simulink model "tsc_lazo_cerrado"  (R2024a)
settings: Solver=ode15s  StartTime=0.0  StopTime=tm_final  MaxStep=tm_h  RelTol=1e-9  AbsTol=1e-11
model workspace (MAT data in the model file):
  tm_C1 = 1.87501784269e-05
  tm_C2 = 3.75003568539e-05
  tm_Cp = 2.89288467158e-06
  tm_L1 = 0.26018031666
  tm_L2 = 0.13009015833
  tm_R1 = 1.15690788571
  tm_R2 = 0.578453942857
  tm_Rb1 = 84640
  tm_Rb2 = 42320
  tm_Rp = 2.20064
  tm_a1 = 1
  tm_a2 = 0.03
  tm_a3 = 0.03
  tm_carga = [0 1e-05 2e-05 3e-05 4e-05 5e-05 6e-05 7e-05 8e-05 9e-05 0.0001 0.00011 ... (160002 elements, 80001x2)]
  tm_final = 0.8
  tm_h = 2.5e-05
  tm_lambda = 229.793279031
  tm_omega = 314.159265359
  tm_vC10 = 0
  tm_vC20 = 0
  tm_vCp0 = 344.473571203
  tsc_cfg.p.L_H = [0.26018031666 0.13009015833]
  tsc_cfg.p.C_F = [1.87501784269e-05 3.75003568539e-05]
  tsc_cfg.p.R_ohm = [1.15690788571 0.578453942857]
  tsc_cfg.p.Rb_ohm = [84640 42320]
  tsc_cfg.p.Cp_F = 2.89288467158e-06
  tsc_cfg.p.Rp_ohm = 2.20064
  tsc_cfg.p.omega = 314.159265359
  tsc_cfg.p.T = 0.02
  tsc_cfg.p.lambda = 229.793279031
  tsc_cfg.p.k = 42.32
  tsc_cfg.p.coefTension = [1 0.03 0.03]
  tsc_cfg.p.limiteDiDt_A_s = 2500
  tsc_cfg.p.limiteDiDtPlan_A_s = 2475
  tsc_cfg.p.margenDiDt = 0.01
  tsc_cfg.p.permanenciaMin_s = 0.06
  tsc_cfg.p.histeresis_A2 = 0.025
  tsc_cfg.p.pasoMuestreo_s = 0.00031746031746
  tsc_cfg.p.ruidoSigma_A = 0
  tsc_cfg.p.PNominal_W = 1000
  tsc_cfg.p.opciones.CasoTension = "moderada"
  tsc_cfg.p.opciones.Modo = "ga"
  tsc_cfg.p.opciones.BitsFijos = [1 0]
  tsc_cfg.p.opciones.PNominal_W = 1000
  tsc_cfg.p.opciones.Duracion_s = 0.8
  tsc_cfg.p.opciones.PasoMaximo_s = 2.5e-05
  tsc_cfg.p.opciones.VCInicial_V = [0 0]
  tsc_cfg.p.opciones.MaxDiDt_A_s = 2500
  tsc_cfg.p.opciones.Permanencia_s = 0.06
  tsc_cfg.p.opciones.Histeresis_A2 = 0.025
  tsc_cfg.p.opciones.MargenDiDt = 0.01
  tsc_cfg.p.opciones.EscalaCarga = [0.45 1.35 0.55 1.15]
  tsc_cfg.p.opciones.InstantesCarga_s = [0 0.2 0.4 0.6]
  tsc_cfg.p.opciones.Transicion_s = 0.06
  tsc_cfg.p.uReferencia = [344.475378053; 342.234056862; 335.572294082; 324.672808973; 309.827507389; 291.419626131; 269.900805928; 245.76494729; 219.520945261; 191.666460359; 162.664759213; 132.926361149; 102.796783137; 72.5511245888; 42.3956243918; 12.4757090319; -17.1105133821; -46.2948235646; -75.0193622969; -103.216997622; -130.793561892; -157.613734298; -183.491988067; -208.189539599; -231.417673404; -252.847222623; -272.123413738; -288.884787089; -302.784526411; -313.512304625; -320.814699368; -324.512354836; -324.512354836; -320.814699368; -313.512304625; -302.784526411; -288.884787089; -272.123413738; -252.847222623; -231.417673404; -208.189539599; -183.491988067; -157.613734298; -130.793561892; -103.216997622; -75.0193622969; -46.2948235646; -17.1105133821; 12.4757090319; 42.3956243918; 72.5511245888; 102.796783137; 132.926361149; 162.664759213; 191.666460359; 219.520945261; 245.76494729; 269.900805928; 291.419626131; 309.827507389; 324.672808973; 335.572294082; 342.234056862]
  tsc_cfg.p.iCargaReferencia = [6.51182189137; 7.16575638416; 7.73235116479; 8.21110783281; 8.60326005793; 8.91131348924; 9.13853778462; 9.2884553265; 9.3643709259; 9.36898275933; 9.30410728819; 9.17054063334; 8.96806671553; 8.69560948452; 8.35151387567; 7.9339288523; 7.44125698892; 6.87262928743; 6.22836178092; 5.51035213356; 4.72237972346; 3.87028111377; 2.9619836181; 2.00739188717; 1.01813500096; 0.00719333849221; -1.01156551506; -2.02390524428; -3.01575305312; -3.97370466865; -4.88546429102; -5.74018819674; -6.52870990668; -7.24363587413; -7.87931251943; -8.43167705693; -8.89801487251; -9.27665428601; -9.56663464748; -9.76738541319; -9.87845198541; -9.89929885692; -9.8292124672; -9.66731590084; -9.41269608903; -9.0646325672; -8.62290617078; -8.08815730582; -7.46225743332; -6.74865473042; -5.95265581387; -5.08160988616; -4.14496932337; -3.15421090963; -2.12261374764; -1.06490229599; 0.00322510035915; 1.06565147543; 2.10644175202; 3.11044532539; 4.06385658961; 4.95469208973; 5.77314935733]
  tsc_cfg.p.cpReferencia = [0.000821056838438 -0.0399433156679 -0.0796021803624 -0.11709608866 -0.151499211358 -0.182073153192 -0.208305554993 -0.229930479172 -0.246929145209 -0.259511271415 -0.268078939042 -0.273176379618 ... (126 elements, 63x2)]
  tsc_cfg.p.x0 = [0; 0; 0; 0; 0; 0]
  tsc_cfg.p.bits = [0  0; 0  1; 1  0; 1  1]
  tsc_cfg.D63 = [0 -10.0309181665 5.02170145378 -3.3547530699 2.52339001873 -2.02628170292 1.69632306201 -1.46190220008 1.28721732655 -1.15238243548 1.04546960893 -0.958891913625 ... (3969 elements, 63x63)]
  tsc_cfg.Modo = "ga"
  tsc_cfg.BitsFijos = [1 0]
  tsc_cfg.TsSupervision = 0.00031746031746
  tsc_cfg.Duracion_s = 0.8
  tsc_cfg.PasoMaximo_s = 2.5e-05
  tsc_cfg.VCInicial_V = [0 0]
  tsc_cfg.CasoTension = "moderada"
  tsc_cfg.opciones.CasoTension = "moderada"
  tsc_cfg.opciones.Modo = "ga"
  tsc_cfg.opciones.BitsFijos = [1 0]
  tsc_cfg.opciones.PNominal_W = 1000
  tsc_cfg.opciones.Duracion_s = 0.8
  tsc_cfg.opciones.PasoMaximo_s = 2.5e-05
  tsc_cfg.opciones.VCInicial_V = [0 0]
  tsc_cfg.opciones.MaxDiDt_A_s = 2500
  tsc_cfg.opciones.Permanencia_s = 0.06
  tsc_cfg.opciones.Histeresis_A2 = 0.025
  tsc_cfg.opciones.MargenDiDt = 0.01
  tsc_cfg.opciones.EscalaCarga = [0.45 1.35 0.55 1.15]
  tsc_cfg.opciones.InstantesCarga_s = [0 0.2 0.4 0.6]
  tsc_cfg.opciones.Transicion_s = 0.06
  tsc_cfg.CargaExogena = [0 1e-05 2e-05 3e-05 4e-05 5e-05 6e-05 7e-05 8e-05 9e-05 0.0001 0.00011 ... (160002 elements, 80001x2)]
  tsc_cfg.vCp0 = 344.473571203
  tsc_cfg.alcance = "Solo simulacion; fuente impuesta, carga sintetica, valvula idealizada, L/C fijos. Control calculado en Simulink durante la ejecucion."
(part 1 of 2)
Description:
  | Simulacion de lazo cerrado: supervisor temporal discreto, ejecutor con deteccion continua de corriente cero y planta RC+2LC con perdidas. No lee cronogramas externos ni llama al motor MATLAB. Fuente impuesta y carga sintetica exogena. Valvula bidireccional idealizada; no SCR fisico. El feedback de control usa Memory (un paso mayor del solver).
settings Model: Creator=paco  LastModifiedBy=paco
settings DataIOCC: SaveOutput=off  SignalLogging=off  SaveTime=off
settings DebuggingCC: AlgebraicLoopMsg=error

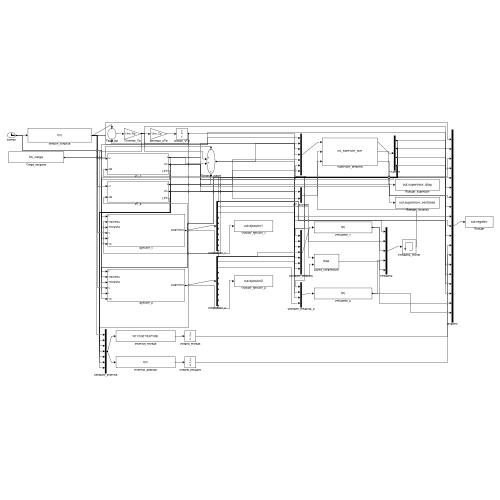
[thumbnail: Simulink's stored preview of the top-level diagram]
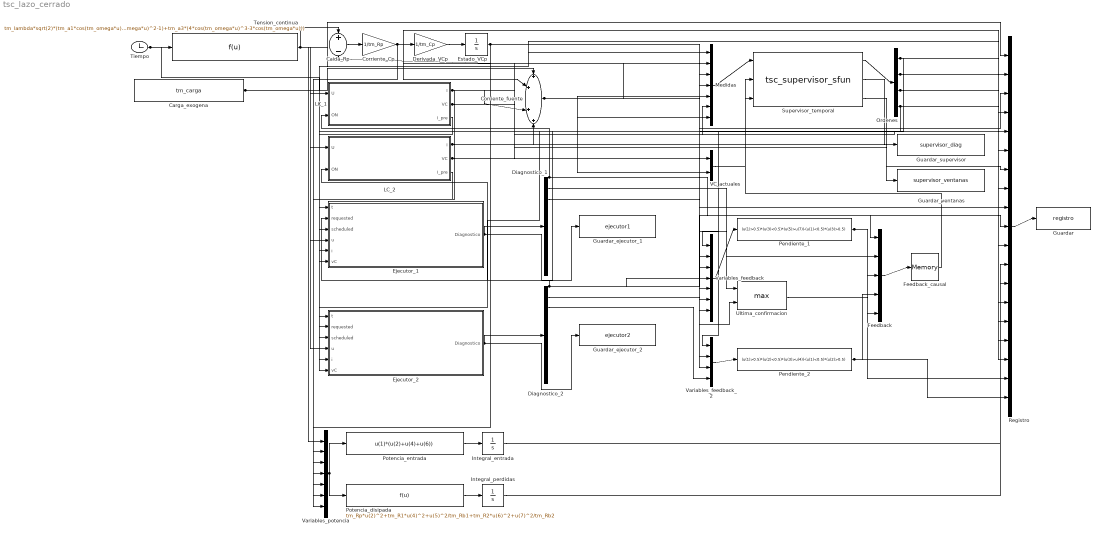
== system tsc_lazo_cerrado ==
  Caida_Rp : Sum  Inputs=+-
  Carga_exogena : FromWorkspace  VariableName=tm_carga  OutputAfterFinalValue=Holding final value
  Corriente_Cp : Gain  Gain=1/tm_Rp
  Corriente_fuente : Sum  Inputs=++++
  Derivada_VCp : Gain  Gain=1/tm_Cp
  Diagnostico_1 : Demux  Outputs=10
  Diagnostico_2 : Demux  Outputs=10
  Ejecutor_1 : Subsystem
  Ejecutor_2 : Subsystem
  Estado_VCp : Integrator  InitialCondition=tm_vCp0
  Feedback : Mux  Inputs=5
  Feedback_causal : Memory  InitialCondition=[0;0;0;0;-1e6]
  Guardar : ToWorkspace  VariableName=registro  SaveFormat=Timeseries  SampleTime=-1
  Guardar_ejecutor_1 : ToWorkspace  VariableName=ejecutor1  SaveFormat=Timeseries  SampleTime=-1
  Guardar_ejecutor_2 : ToWorkspace  VariableName=ejecutor2  SaveFormat=Timeseries  SampleTime=-1
  Guardar_supervisor : ToWorkspace  VariableName=supervisor_diag  SaveFormat=Timeseries  SampleTime=tsc_cfg.TsSupervision
  Guardar_ventanas : ToWorkspace  VariableName=supervisor_ventanas  SaveFormat=Timeseries  SampleTime=tsc_cfg.p.T
  Integral_entrada : Integrator
  Integral_perdidas : Integrator
  LC_1 : Subsystem
  LC_2 : Subsystem
  Medidas : Mux  Inputs=7
  Ordenes : Demux
  Pendiente_1 : Fcn  Expr=(u(1)>0.5)*(u(3)<0.5)*(u(5)>u(7))-(u(1)<0.5)*(u(3)>0.5)
  Pendiente_2 : Fcn  Expr=(u(1)>0.5)*(u(2)<0.5)*(u(3)>u(4))-(u(1)<0.5)*(u(2)>0.5)
  Potencia_disipada : Fcn  Expr=tm_Rp*u(2)^2+tm_R1*u(4)^2+u(5)^2/tm_Rb1+tm_R2*u(6)^2+u(7)^2/tm_Rb2
  Potencia_entrada : Fcn  Expr=u(1)*(u(2)+u(4)+u(6))
  Registro : Mux  Inputs=19
  Supervisor_temporal : M-S-Function  FunctionName=tsc_supervisor_sfun  Parameters=tsc_cfg
  Tension_continua : Fcn  Expr=tm_lambda*sqrt(2)*(tm_a1*cos(tm_omega*u)+tm_a2*(2*cos(tm_omega*u)^2-1)+tm_a3*(4*cos(tm_omega*u)^3-3*cos(tm_omega*u)))
  Tiempo : Clock
  Ultima_confirmacion : MinMax  Function=max  Inputs=2
  VC_actuales : Mux  Inputs=2
  Variables_feedback : Mux  Inputs=7
  Variables_feedback_2 : Mux
  Variables_potencia : Mux  Inputs=7
  wires:
  Tiempo/1 -> Tension_continua/1, Ejecutor_1/1(t), Ejecutor_2/1(t)
  Tension_continua/1 -> Caida_Rp/1, LC_1/1(U), Ejecutor_1/4(u), LC_2/1(U), Ejecutor_2/4(u), Medidas/1, Variables_potencia/1, Registro/1
  Estado_VCp/1 -> Caida_Rp/2, Variables_potencia/3, Registro/5
  Caida_Rp/1 -> Corriente_Cp/1
  Corriente_Cp/1 -> Derivada_VCp/1, Corriente_fuente/2, Medidas/3, Variables_potencia/2, Registro/4
  Derivada_VCp/1 -> Estado_VCp/1
  Carga_exogena/1 -> Corriente_fuente/1, Registro/2
  Diagnostico_1/1 -> LC_1/2(ON), Variables_feedback/3, Feedback/1, Registro/10
  LC_1/1(I) -> Corriente_fuente/3, Medidas/4, Variables_potencia/4, Registro/6
  Ordenes/1 -> Ejecutor_1/2(requested), Variables_feedback/1, Registro/14
  Ordenes/3 -> Ejecutor_1/3(scheduled), Variables_feedback/5, Registro/16
  LC_1/3(I_pre) -> Ejecutor_1/5(i)
  LC_1/2(VC) -> Ejecutor_1/6(vC), Medidas/6, VC_actuales/1, Variables_potencia/5, Registro/7
  Ejecutor_1/1(Diagnostico) -> Diagnostico_1/1, Guardar_ejecutor_1/1
  Diagnostico_2/1 -> LC_2/2(ON), Variables_feedback/4, Variables_feedback_2/2, Feedback/2, Registro/11
  LC_2/1(I) -> Corriente_fuente/4, Medidas/5, Variables_potencia/6, Registro/8
  Ordenes/2 -> Ejecutor_2/2(requested), Variables_feedback/2, Variables_feedback_2/1, Registro/15
  Ordenes/4 -> Ejecutor_2/3(scheduled), Variables_feedback/6, Variables_feedback_2/3, Registro/17
  LC_2/3(I_pre) -> Ejecutor_2/5(i)
  LC_2/2(VC) -> Ejecutor_2/6(vC), Medidas/7, VC_actuales/2, Variables_potencia/7, Registro/9
  Ejecutor_2/1(Diagnostico) -> Diagnostico_2/1, Guardar_ejecutor_2/1
  Corriente_fuente/1 -> Medidas/2, Registro/3
  Medidas/1 -> Supervisor_temporal/1
  Feedback_causal/1 -> Supervisor_temporal/2
  VC_actuales/1 -> Supervisor_temporal/3
  Supervisor_temporal/1 -> Ordenes/1
  Supervisor_temporal/2 -> Guardar_supervisor/1
  Supervisor_temporal/3 -> Guardar_ventanas/1
  Diagnostico_1/3 -> Variables_feedback/7
  Diagnostico_2/3 -> Variables_feedback_2/4
  Variables_feedback/1 -> Pendiente_1/1
  Variables_feedback_2/1 -> Pendiente_2/1
  Diagnostico_1/2 -> Ultima_confirmacion/1
  Diagnostico_2/2 -> Ultima_confirmacion/2
  Pendiente_1/1 -> Feedback/3, Registro/18
  Pendiente_2/1 -> Feedback/4, Registro/19
  Ultima_confirmacion/1 -> Feedback/5
  Feedback/1 -> Feedback_causal/1
  Variables_potencia/1 -> Potencia_entrada/1, Potencia_disipada/1
  Potencia_entrada/1 -> Integral_entrada/1
  Potencia_disipada/1 -> Integral_perdidas/1
  Integral_entrada/1 -> Registro/12
  Integral_perdidas/1 -> Registro/13
  Registro/1 -> Guardar/1
